simulink model "EV6_LUT_FourWheel_EV6Battery77p4kWh_PowerCorrected"  (R2024a)
settings: Solver=ode4  StartTime=0  StopTime=60  FixedStep=0.001  RelTol=1e-3
PreLoadFcn:
  | VSS_BICYCLE=Simulink.Variant('Dual=0');
  | VSS_DUAL=Simulink.Variant('Dual=1');
  | Dual=1;
  | load('DriveCycle2.mat')
PostLoadFcn:
  | if any(exist('dsrtsu_mdlpostloadfcn', 'file') ~= 0), dsrtsu_mdlpostloadfcn('Execute', bdroot); end
InitFcn:
  | , if any(exist('rtifpga_mdlclblib', 'file') ~= 0), rtifpga_mdlclblib('Init', bdroot); end,
  | , if any(exist('dsmpb_private', 'file') ~= 0), dsmpb_private('dsmpb_mdlclblib', 'Init', bdroot); end,
  | load('DriveCycle2.mat')
model workspace (MAT data in the model file):
  DiffRatio = 10.65
  EV6_2023_BattBranchCapacity_Ah = 55.5236728838
  EV6_2023_BattEnergy_kWh = 77.4
  EV6_2023_BattNominalVoltage_V = 697
  EV6_2023_BattNumCellsParallel = 2
  EV6_2023_BattNumCellsSeries = 192
  EV6_2023_BattOpenVoltCapBpts = [0 0.1 0.2 0.3 0.4 0.5 0.6 0.7 0.8 0.9 1]
  EV6_2023_BattOpenVoltTbl = [2.96762142548 3.40364281191 3.47417488548 3.54470541822 3.61523441014 3.68576186124 3.75628777151 3.82681214095 3.94527005036 4.07101207308 4.2120755254]
  EV6_2023_BattPackCapacity_Ah = 111.047345768
  EV6_2023_BattResistSocBpts = [0 0.2 0.4 0.6 0.8 1]
  EV6_2023_BattResistTbl = [0.0163620057716  0.0172368903217  0.0166967924599  0.0156665372921  0.0190883901835  0.0243044037801; 0.0118174152018  0.0121226074867  0.0102711076249  0.010219317419  0.0111774362286  0.0144365199014; 0.00807187352333  0.00758541551769  0.00750957985901  0.00638499253037  0.00711375471373  0.0083548700057; 0.00375663957972  0.00474065349228  0.00468331433572  0.00455013952048  0.00502364997465  0.00563588419468; 0.00266904525531  0.00337561163613  0.00332012212978  0.00328867807619  0.00355872700708  0.00413211857267; 0.00103635901355  0.00133026843217  0.00127385410071  0.00139778066489  0.00136041773062  0.00187554531454; 0.0019014404175  0.00247483198309  0.00184965021158  0.00284106272499  0.0028595592271  0.00515867444009]
  EV6_2023_BattResistTempBpts = [243.1 253.1 263.1 273.1 283.1 298.1 313.1]
  EV6_2023_InitialPackOCV_V = 726.471714233
  EV6_2023_InitialSOC = 0.638878863672
  EV6_BattCellCapacity_Ah = 60.3
  EV6_BattInitialSOC = 0.638878863672
  EV6_BattOCV_Cell_V = [2.96762142548 3.40364281191 3.47417488548 3.54470541822 3.61523441014 3.68576186124 3.75628777151 3.82681214095 3.94527005036 4.07101207308 4.2120755254]
  EV6_BattOCV_SOC = [0 0.1 0.2 0.3 0.4 0.5 0.6 0.7 0.8 0.9 1]
  EV6_BattPackCapacity_Ah = 120.6
  EV6_BattParallelCells = 2
  EV6_BattResistanceSOC = [0 0.2 0.4 0.6 0.8 1]
  EV6_BattResistanceTable_Ohm = [0.0163620057716  0.0172368903217  0.0166967924599  0.0156665372921  0.0190883901835  0.0243044037801; 0.0118174152018  0.0121226074867  0.0102711076249  0.010219317419  0.0111774362286  0.0144365199014; 0.00807187352333  0.00758541551769  0.00750957985901  0.00638499253037  0.00711375471373  0.0083548700057; 0.00375663957972  0.00474065349228  0.00468331433572  0.00455013952048  0.00502364997465  0.00563588419468; 0.00266904525531  0.00337561163613  0.00332012212978  0.00328867807619  0.00355872700708  0.00413211857267; 0.00103635901355  0.00133026843217  0.00127385410071  0.00139778066489  0.00136041773062  0.00187554531454; 0.0019014404175  0.00247483198309  0.00184965021158  0.00284106272499  0.0028595592271  0.00515867444009]
  EV6_BattResistanceTemp_K = [243.1 253.1 263.1 273.1 283.1 298.1 313.1]
  EV6_BattSeriesCells = 192
  EV6_FinalDriveRatio = 10.65
  EV6_TargetPackResistance_Ohm = 0.132763804608
  Gas = 0.383333333333
undefined symbols (not defined in the file): accel_bp_mps2, AccelCmd, ActTqLF_Nm_, ActTqLR_Nm_, ActTqRF_Nm_, ActTqRR_Nm_, BattChargeLimitMaxPwr, BattChargeLimitSocBpts, BattChargeLimitTbl, BattDischargeLimitSocBpts, BattDischargeLimitTbl, BattDischargeMaxPwr, BrakeMaxPrs, BrakeMaxTrq, ChassisDistCg2FrontAxle, ChassisDistCg2RearAxle, ChassisVehMass, CltchCmd, CoastDown, DecelCmd, DiscIntNeverNeededParam, EnvGravCnst, EnvPrs, EnvTemp, EV6_RegenTorqueGain, EV6_TractionTorqueGain, front_share_regen_3d, front_share_traction_3d, FuelSpecificGrav, GearCmd, h, InitStates, lgSw, limitedMCT, MCT, MtrEffSpdBpts, MtrEffTbl, MtrEffTrqBpts, MtrPwrMax, MtrTrqMax, out_1, pMCT, RealSimPara, Ref_speed, Ref_time, regen_torque_bp_Nm, speed_bp_kph, SteeringCmd, SupvsryCtrlRegenBrkCutOffTbl, SupvsryCtrlRegenSpdBpts, TestScnrioCycleNum, traction_torque_bp_Nm, US06, VEH
libraries: VSIGenLib x65, simulink x54, etargetslib x38, dsmpblib x24, vehdynlibtire x12, autolibshared x11, vehdynlibsuspension x7, vehdynlibtirecommon x7, autolibpowerinfoutils x6, autolibutils x5, autolibsharedcoupling x4, autolibmappedmotor x4
(part 1 of 19)
PreSaveFcn:
  | , if any(exist('dsmpb_private', 'file') ~= 0), dsmpb_private('dsmpb_mdlclblib', 'PreSave', bdroot); end,
CloseFcn:
  | , if any(exist('dsmpb_private', 'file') ~= 0), dsmpb_private('dsmpb_mdlclblib', 'Close', bdroot); end,
settings Model: DataDictionary=DdPassengerEv.sldd  DSMPB_ID_DATA={'18088',struct('BlockId','f88c42c2-e70e-4436-bd85-ff34452e836e','SignalIds',{{'1df572a0-f117-4729-9091-2c1a0a26ec90','0824b86c-995c-4624-95de-4f5a118cf0f7','1af539eb-325a-4e38-9107-84d6b0267392','ebb0fa34-559f-4fe0-b409-8a817ae8753c','d7145080-d35d-4c02-8c9e-cf76ffb14dc2','5075bfde-4142-4aeb-b309-025b37120541','abbab0bd-1456-4252-a37b-ee5f55ea0579','b5d617b8-bb24-4539-9145-e591a0a295f8','7df03788-1936-4801-98c0-dd7f6dfcacba','19949bfb-f246-4995-90e8-29a3751a0fa7','9454b59a-aedd-4270-89a6-1cca43305823','37cf720c-23c2-4b6d-8589-7b035c806643','98db9f76-eafd-4d54-90d2-d997d73b87d4','ff589fc8-5b21-4798-a75e-d26fc35c1fa1','e61b2882-e27e-4f06-b730-5e5281621b34','6605e0e6-8bf3-4a45-a0b0-4b9c1cf463f3','0d0f5161-daad-47a1-bb1d-ec2adbc183ca','48ba6675-0966-4a1c-b127-4f76dca3de94','3c897f11-b2eb-4eb8-b88f-7b7e913c6e41','378f468e-364f-43c5-91f9-fc8ddef6aca6','9c7f20ac-956d-4c19-bdea-31a2a3930ea2','bc252920-9c7c-4b91-a017-ee1d69e3f03c','a5e7a104-8664-4690-a58a-7cbf05737866','fe1cfa34-9b23-4225-85e3-0403f07d36e7','ab40d80a-815e-4994-aacd-e42d283f5b3a','2a4143b2-c438-4d42-997d-0587141eb8f0','2686c37a-8724-40b3-99fb-f8873ba286b8','3707aa1b-88c1-4f14-8f25-f346aa75c252','7413af4b-f834-4020-ad34-3dd98c546e0c','3445835b-9a90-4408-a32d-d76b66b0385b','23c9a144-1259-4fa3-9a16-4a32a7eadff9','5b4206b0-ea89-4111-86f7-7a4fd8c76b72','85c84ea6-72b6-4ccb-9199-727b305580c3','97bb0073-9d03-44a9-972d-49a0eb465678','8c3f0698-b0b6-4624-aa00-3a3096f7cc2f','c968922f-253e-433f-ad46-daf21e902962','21ad150a-19dc-415b-bc1b-b39528ec9221','a3572415-9467-4ff8-a492-c6c1b3cb1b64','700ac678-fb53-40b6-8e97-9eeffe7a1ca8','14ed5f8b-aa1d-402b-b493-5622a729893d','bdbcc0b3-c6a4-485e-8fbf-8c12a8df89e7','7a19cc2b-f06b-466f-ae52-fb8ac6fb0258','87deda6a-2251-4462-8ae0-a20845c776d4','41874d9b-304a-4265-a3a1-69d5c58383ea'}}),'18719',struct('BlockId','79daabbd-4df4-4017-ba65-d977f7e6cd2f','SignalIds',{{'63c99320-3a8a-469e-8a50-5c577229603f'}}),'18720',struct('BlockId','9f21d727-31d5-41b9-aed1-27a40d8edf8b','SignalIds',{{'abab19c9-0d91-46eb-acba-2a4710e305d8'}}),'18721',struct('BlockId','5513e588-accc-447f-8233-209349c29c53','SignalIds',{{'cf7c35a9-6bda-4f5f-bfb5-f51ad44c376b'}}),'18722',struct('BlockId','a427ee23-ff95-4a9c-807f-ad2b61c33ee4','SignalIds',{{'b3e368f1-9670-4dd7-aa42-1fcccca64ddf'}}),'18723',struct('BlockId','53805a71-03ad-4b45-a2ab-66e4ec3700d0','SignalIds',{{'0801da20-d997-46db-8512-e37e1180e77c','d193450d-1a5a-4c8d-a2ac-d5fd306fefe3'}}),'18724',struct('BlockId','4d4909f9-4869-4ae2-8541-060fc5e29366','SignalIds',{{'0588d1ac-5d02-4ce0-9f56-5f4e572c1088','c0609b3e-104e-46bb-beb6-dc1d54d218ce','a0011887-c3f0-4769-95be-c916ccb77447','feb7a80d-e7d1-407d-8b44-49f086fb9d8a'}}),'27205',struct('BlockId','7f292e34-acca-4213-92cf-eac8a4e11745','SignalIds',{{'6a46899f-e089-4ce6-a50d-bdb6920dc331'}}),'27206',struct('BlockId','0e302573-500f-4275-88ba-9cf54fc32ddf','SignalIds',{{'b049b44b-cb75-4882-8bfb-1e055380ad24'}}),'27207',struct('BlockId','894fc26a-3344-4696-abb1-a58f33cf2fe5','SignalIds',{{'56006949-e5f9-49a3-9093-d3c1068f762e'}}),'27282',struct('BlockId','99a4c3a2-8dee-4bd9-95aa-231a7d48a6ad','SignalIds',{{'ad35807f-d183-4bfc-ba2d-784a27a526e2'}}),'27283',struct('BlockId','c3bde5a4-346e-4338-b541-b63d4485ff5c','SignalIds',{{'fd571466-ead4-4f47-b3e3-1d8d73dd83aa'}}),'27284',struct('BlockId','f9cc58a0-b533-4fcd-ba24-c41d1087025b','SignalIds',{{'edc79761-e8e8-4577-bee1-99dd85130da2'}}),'27290',struct('BlockId','912f2a14-bc8b-461e-a925-b64698223e59','SignalIds',{{'776489e0-d1be-4c01-975d-6bf488838e0f'}}),'27291',struct('BlockId','568bb84e-3e6c-4e27-b5f8-f420efc72c29','SignalIds',{{'ed34b8f1-74db-4d36-9a75-d105186c40b5'}}),'27292',struct('BlockId','c169ab68-0334-4d5e-8995-fe0588a530be','SignalIds',{{'fac7e22a-c9c5-48bf-8dd3-1207989a75ce'}}),'27321',struct('BlockId','486c1cde-04a2-4a7b-bb1b-0ecc89f4c4dc','SignalIds',{{'92ff9d42-6575-4421-bf12-cd2858422bf3'}}),'27322',struct('BlockId','3f4e80df-9a0c-4630-abed-705861a8f37f','SignalIds',{{'ecbbb69e-a9c9-45ac-a3ac-ebec06b4c832'}}),'27830',struct('BlockId','3345bd5a-57a2-4283-ba1f-19d9b3e140a9','SignalIds',{{'92c21d5f-d0b1-43b1-b6bc-24cdf5ae3b2f'}}),'27838',struct('BlockId','d4a4d4a9-28f7-4103-93fc-48b8f34cb05d','SignalIds',{{'869cfc04-7b3a-4508-9a04-d408d22a8585','a495f60b-e320-4589-a7da-c9c1e0fb9d66','cadd7efe-3805-4998-94fe-0c2d1fc01ff7','5d968b47-a87d-4eb2-a743-bf289ed725ef','78d13881-677a-4003-a1ce-a7b3fd4b10ed'}}),'27839',struct('BlockId','a8a28146-2bd5-46fa-a2eb-22a81d10cc62','SignalIds',{{'0cba0fcf-c449-40bd-9ed4-ab01110a305a','4e2eaeac-0381-4090-a698-3e33368cf49b'}}),'27843',struct('BlockId','b81313f3-c14d-43f5-aca0-17ec7f04c03a','SignalIds',{{'c33cb8ae-acba-4ded-b0d5-2f0e98182df7'}}),'28333',struct('BlockId','b4192faa-dd44-47ab-a57b-d849e8842c53','SignalIds',{{'3c64dc78-c053-4e1d-a3dc-7d922541f734'}}),'28409',struct('BlockId','364dbf1f-db94-48e0-9add-af905e700009','SignalIds',{{'403b6449-3746-476e-bb2d-b20219d4f4bb','7d755994-2bec-4eab-9fef-7bc71a1fff8b','73ba929b-0017-4bba-a1b8-b6b44c7091ab','1b99e985-b5b3-4b9e-96cf-f375f8e62d9c','ea9d5c72-c4df-42a7-a1b2-83c8aa561c19'}})}  RTICANMMDATA=struct('GeneralSetupData',struct('modelroot','C:\GitDev\Anye\cave_carla_dev\Vehicles\VehicleProjects\Bolt_EV\System','generalsettings',struct('filesettings',struct('destfolder',struct('Name','RTICANMM_FILES','Check',1),'buildfolder',struct('Name','.','Check',1),'AbsDestfolder',struct('Name','C:\GitDev\Anye\cave_carla_dev\Vehicles\VehicleProjects\Bolt_EV\System\RTICANMM_FILES'),'AbsBuildfolder',struct('Name','C:\GitDev\Anye\cave_carla_dev\Vehicles\VehicleProjects\Bolt_EV\System'))),'options',struct('addpaths',1,'rmpaths',1,'addtrcexclusion',true,'cannavigator',struct('checkmonitoring',0),'show_usrtrc',0,'use_usrtrc',0),'advanced',struct('options',ones(1,100)),'MPSetup',{{}},'RTI',struct('Type','DSRT','Ver','4.2p1','Date','11-Feb-2020'),'modelname','CAVE_MachE','block','CAVE_MachE'))  DSRTSU_INTERNAL_RTIFPGA=210  DSRTSU_INTERNAL_RTISTBM_VER=24.1  PauseTimes=45  Creator=9bt  LastModifiedBy=ssl35511
settings SolverCC: AlgebraicLoopSolver=TrustRegion
settings OptimizationCC: BlockReduction=off  ConditionallyExecuteInputs=off  OptimizeBlockIOStorage=off  BufferReuse=off  GlobalBufferReuse=off  ExpressionFolding=off  LocalBlockOutputs=off  OptimizeDataStoreBuffers=off  BusAssignmentInplaceUpdate=off
settings DebuggingCC: MergeDetectMultiDrivingBlocksExec=none  TasksWithSamePriorityMsg=none  ParameterOverflowMsg=none  ParameterUnderflowMsg=error  UnconnectedInputMsg=warning  UnconnectedOutputMsg=warning  UnconnectedLineMsg=warning  UnderSpecifiedDimensionMsg=warning
settings HardwareCC: ProdBitPerLong=64  ProdLargestAtomicInteger=Integer  ProdWordSize=32  ProdHWDeviceType=Custom Processor->Custom
settings ModelReferenceCC: EnableRefExpFcnMdlSchedulingChecks=on  PropagateSignalLabelsOutOfModel=off
settings SFSimCC: MATLABDynamicMemAlloc=off
settings RTWCC: Description=dSPACE Run-Time Target (for VEOS on Windows and ConfigurationDesk)  SystemTargetFile=dsrt.tlc  GenCodeOnly=on  MakeCommand=make_dsrt  TemplateMakefile=dsrt_default_tmf  RTWVerbose=off  GPUComputeCapability=3.5
settings CodeAppCC: MaxIdLength=63  StateflowObjectComments=on
settings STFCustomTargetCC: ParMdlRefBuildCompliant=on  GRTInterface=off  UseToolchainInfoCompliant=off  SystemTargetFile=dsrt.tlc
settings GRTTargetCC: CompOptLevelCompliant=off  ConcurrentExecutionCompliant=off  CombineOutputUpdateFcns=off  MatFileLogging=off  CPPClassGenCompliant=off  UseToolchainInfoCompliant=off

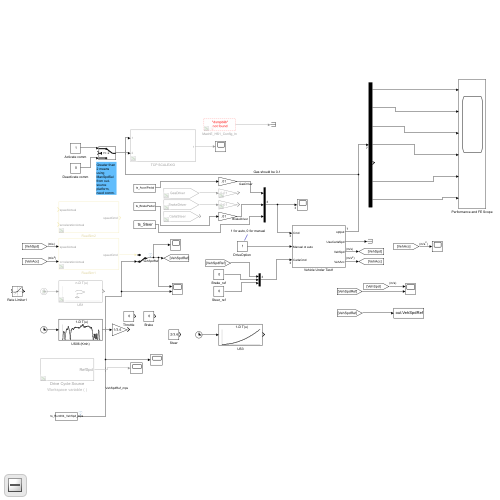
[thumbnail: Simulink's stored preview of the top-level diagram]
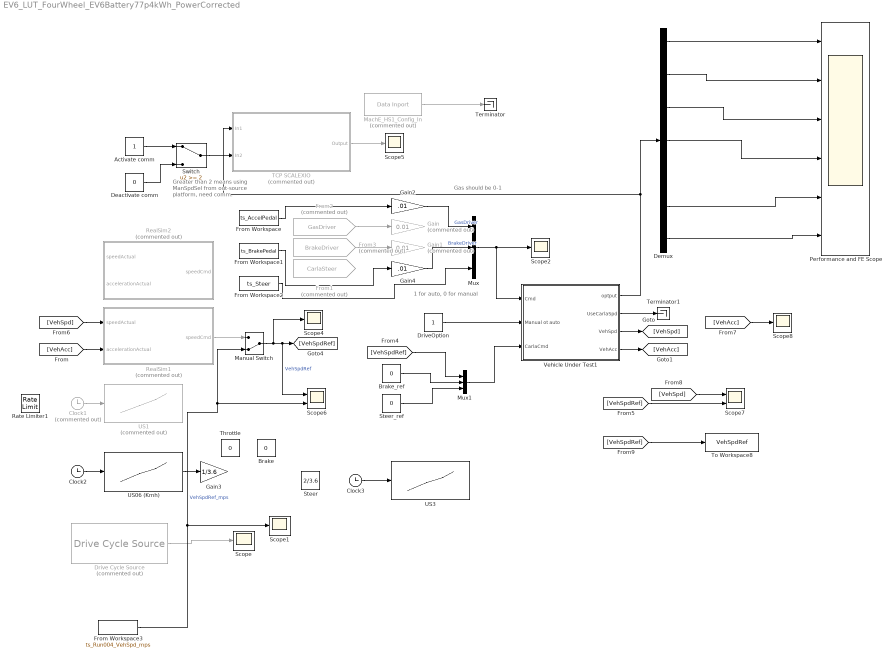
== system EV6_LUT_FourWheel_EV6Battery77p4kWh_PowerCorrected ==
  note: Greater than 2 means using ManSpdSel from out-source platform, need comm.
  note: 1 for auto, 0 for manual
  note: Gas should be 0-1
  Activate comm : Constant
  Brake : Constant  Value=0
  Brake_ref : Constant  Value=0
  Clock1 : Clock  Commented=on
  Clock2 : Clock
  Clock3 : Clock
  Deactivate comm : Constant  Value=0
  Demux : Demux  Outputs=7
  Drive Cycle Source : autolibshared/Drive Cycle Source  Commented=on  cycleVar=Workspace variable  wsVar=spd_kmh_ts  fileVar=cycleFTP75.mat  tfinal=""  cycleRepeat=off  outAccPort=off  outGearPort=off  gearList=No gear data  t_wot1=5  xdot_woto=0  xdot_wot1=30  t_wot2=20  xdot_wot2=0  t_wotend=30  srcUnit=km/h  outUnit=km/h  srcAccUnit=m/s/s  outAccUnit=m/s^2  dt=0  aMode=1  faultOption=off  velBnd=2  velBndUnit=mph  inUnit=m/s  timeBnd=1  failOption=off  stopSim=off  maxFaultCnt=10  maxFaultTime=2  maxTotFaultTime=15  traceOption=off  dtTrace=1  traceWindow=10  lastDCname=Custom Data Set 1  lastOutUnit=mph  lastDT=0  lastTB=1  lastSB=2  forceCalcBound=off
  DriveOption : Constant
  From Workspace : FromWorkspace  VariableName=ts_AccelPedal
  From Workspace1 : FromWorkspace  VariableName=ts_BrakePedal
  From Workspace2 : FromWorkspace  VariableName=ts_Steer
  From Workspace3 : FromWorkspace  VariableName=ts_Run004_VehSpd_mps
  From1 : From  Commented=on  GotoTag=CarlaSteer  TagVisibility=global
  From2 : From  Commented=on  GotoTag=GasDriver  TagVisibility=global
  From3 : From  Commented=on  GotoTag=BrakeDriver  TagVisibility=global
  Gain : Gain  Commented=on  Gain=0.01
  Gain1 : Gain  Commented=on  Gain=0.01
  Gain2 : Gain  Gain=.01
  Gain3 : Gain  Gain=1/3.6
  Gain4 : Gain  Gain=.01
  MachE_HS1_Config_In : dsmpblib/Data Inport  Priority=10000  Commented=on
      settings: SourceProductName=dSPACE Model Interface Package for Simulink (MIPS)
  Manual Switch : ManualSwitch  CurrentSetting=0
  Mux : Mux  Inputs=3
  Mux1 : Mux  Inputs=3
  Performance and FE Scope : Scope  NumInputPorts=6
  Rate Limiter1 : RateLimiter  RisingSlewLimit=4  FallingSlewLimit=-4  SampleTimeMode=inherited
  RealSim1 : Subsystem  Commented=on
  RealSim2 : Subsystem  Commented=on
  Scope{,1..2,4..5,8} (6 alike) : Scope
  Scope6 : Scope  NumInputPorts=2
  Scope7 : Scope  NumInputPorts=2
  Steer : Constant  Value=2/3.6
  Steer_ref : Constant  Value=0
  Switch : Switch  Threshold=2  SaturateOnIntegerOverflow=off  InputSameDT=off
  TCP SCALEXIO : Subsystem  Commented=on
  Terminator : Terminator
  Terminator1 : Terminator
  Throttle : Constant  Value=0
  To Workspace8 : ToWorkspace  VariableName=VehSpdRef  SaveFormat=Timeseries  SampleTime=0.1
  US06 (Kmh) : Lookup_n-D  NumberOfTableDimensions=1  BreakpointsForDimension1=US06.Time  Table=US06.Speed  InternalRulePriority=Speed  RndMeth=Simplest
  US1 : Lookup_n-D  Commented=on  NumberOfTableDimensions=1  BreakpointsForDimension1=out_1.VehSpdRef.Time  Table=out_1.VehSpdRef.Data  InternalRulePriority=Speed  RndMeth=Simplest
  US3 : Lookup_n-D  NumberOfTableDimensions=1  BreakpointsForDimension1=0:1:100  Table=1/100*[0:1:100].^2  InternalRulePriority=Speed  RndMeth=Simplest
  Vehicle Under Test1 : Subsystem
  wires:
  Mux/1 -> Vehicle Under Test1/1(Cmd), Scope2/1
  DriveOption/1 -> Vehicle Under Test1/2(Manual ot auto)
  From2/1 -> Gain/1
  From3/1 -> Gain1/1
  MachE_HS1_Config_In/1 -> Terminator/1
  Vehicle Under Test1/1(optput) -> TCP SCALEXIO/1(In1), Demux/1
  Switch/1 -> TCP SCALEXIO/2(In2)
  TCP SCALEXIO/1(Output) -> Scope5/1
  Deactivate comm/1 -> Switch/3
  Activate comm/1 -> Switch/1
  Manual Switch/1 -> Scope4/1, Scope6/1, [VehSpdRef]  "VehSpdRef"
  RealSim1/1(speedCmd) -> Manual Switch/1
  [VehAcc] -> RealSim1/2(accelerationActual)
  [VehSpd] -> RealSim1/1(speedActual)
  [VehSpdRef] -> Mux1/1
  Mux1/1 -> Vehicle Under Test1/3(CarlaCmd)
  Vehicle Under Test1/3(VehSpd) -> [VehSpd]
  Vehicle Under Test1/4(VehAcc) -> [VehAcc]
  Steer_ref/1 -> Mux1/3
  Brake_ref/1 -> Mux1/2
  Vehicle Under Test1/2(UseCarlaSpd) -> Terminator1/1
  Clock1/1 -> US1/1
  [VehSpdRef] -> Scope7/2
  Demux/1 -> Performance and FE Scope/1
  Demux/7 -> Performance and FE Scope/6
  Demux/6 -> Performance and FE Scope/5
  Demux/4 -> Performance and FE Scope/4
  Demux/3 -> Performance and FE Scope/3
  Demux/2 -> Performance and FE Scope/2
  [VehAcc] -> Scope8/1
  [VehSpd] -> Scope7/1
  [VehSpdRef] -> To Workspace8/1
  Clock2/1 -> US06 (Kmh)/1
  Clock3/1 -> US3/1
  Drive Cycle Source/1 -> Scope/1
  US06 (Kmh)/1 -> Gain3/1
  From Workspace3/1 -> Scope1/1, Scope6/2, Manual Switch/2  "VehSpdRef_mps"
  From Workspace/1 -> Gain2/1
  Gain2/1 -> Mux/1  "GasDriver"
  From Workspace1/1 -> Gain4/1
  Gain4/1 -> Mux/2  "BrakeDriver"
  From Workspace2/1 -> Mux/3

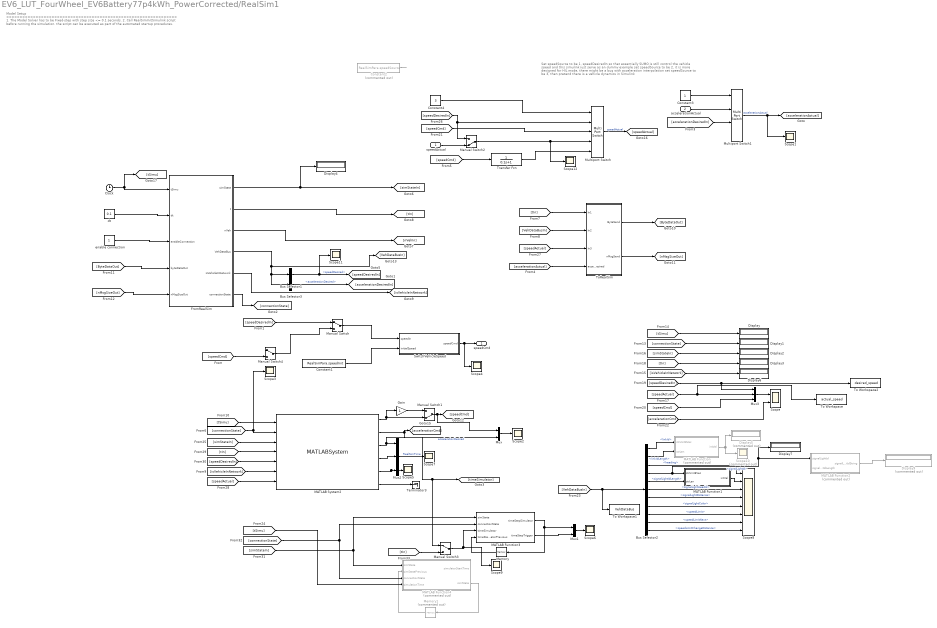
== system EV6_LUT_FourWheel_EV6Battery77p4kWh_PowerCorrected/RealSim1 ==
  note: Set speedSource to be 1, speedDesiredIn so that essentially SUMO is still control the vehicle speed and this simulink just serve as an dummy example
      |
      | set speedSource to be 2, it is more designed for HIL mode, there might be a bug with acceleration interpolation
      |
      | set speedSource to be 3, then pretend there is a vehicle dynamics in Simulink
  note: Model Setup
      | ================================================================
      | 1. The Model Solver has to be Fixed-step with step size <= 0.1 seconds.
      | 2. Call RealSimInitSimulink script before running the simulation. the script can be executed as part of the automated startup procedures.
  speedActual : Inport
  accelerationActual : Inport  Port=2
  Bus Selector1 : BusSelector  OutputSignals=speedDesired
  Bus Selector2 : BusSelector  OutputSignals=linkId,linkIdLength,heading,signalLightId,signalLightIdLength,signalLightHeadId,signalLightDistance,signalLightColor,speedLimit,speedLimitNext,speedLimitChangeDistance
  Bus Selector3 : BusSelector  OutputSignals=accelerationDesired
  Clock : Clock
  Constant1 : Constant  Value=RealSimPara.speedInit
  Constant2 : Constant  Commented=on  Value=RealSimPara.speedSource
  Constant3 : Constant
  Constant4 : Constant  Value=3
  Display{,1..4,6..7} (7 alike) : Display
  Display5 : Display  Commented=on
  Display9 : Display  Commented=on
  FromRealSim : Subsystem
  Gain : Gain
  MATLAB Function : MATLAB Function  Commented=on  TreatAsAtomicUnit=on
  MATLAB Function1 : MATLAB Function  TreatAsAtomicUnit=on
  MATLAB Function2 : MATLAB Function  Commented=on  TreatAsAtomicUnit=on  SystemSampleTime=0.001
  MATLAB Function3 : MATLAB Function  TreatAsAtomicUnit=on
  MATLAB Function4 : MATLAB Function  Commented=on  TreatAsAtomicUnit=on
  MATLAB System2 : MATLABSystem  System=RealSimInterpSpeed  initialSpeed=RealSimPara.speedInit  speedLookAheadHorizon=RealSimPara.tLookahead  speedUpperBound=30  smoothWindow=RealSimPara.smoothWindow  SimulateUsing=Interpreted execution
      mask Type: RealSimInterpSpeed
      mask Display:
      | disp('RealSimInterpSpeed');
      | port_label('input',1,'simulationTime');
      | port_label('input',2,'connectionState');
      | port_label('input',3,'simState');
      | port_label('input',4,'timeReceive');
      | port_label('input',5,'speedReceive');
      | port_label('input',6,'isVehicleInNetwork');
      | port_label('input',7,'speedActual');
      | port_label('output',1,'speedLookAhead');
      | port_label('output',2,'accelerationDesired');
      | port_label('output',3,'timeSimulator');
      | port_label('output',4,'timeStepSimulator');
      | port_label('output',5,'timeStepTrigger');
      | port_label('output',6,'RealSimDelay');
  Manual Switch : ManualSwitch
  Manual Switch1 : ManualSwitch  CurrentSetting=0
  Manual Switch2 : ManualSwitch  CurrentSetting=0
  Manual Switch3 : ManualSwitch
  Manual Switch4 : ManualSwitch
  Memory : Memory
  Memory1 : Memory  Commented=on
  Multiport Switch : MultiPortSwitch  Inputs=4  SaturateOnIntegerOverflow=off  InputSameDT=off
  Multiport Switch1 : MultiPortSwitch  SaturateOnIntegerOverflow=off  InputSameDT=off
  Mux : Mux  Inputs=2
  Mux1 : Mux  Inputs=2
  Mux2 : Mux  Inputs=3
  Mux3 : Mux  Inputs=3
  Scope : Scope  NumInputPorts=2
  Scope{1..7,9,11..12} (10 alike) : Scope
  Scope10 : Scope  Commented=on
  Scope8 : Scope  NumInputPorts=8
  SwitchVehicleSpeed : Subsystem
  Terminator3 : Terminator
  To Workspace : ToWorkspace  VariableName=actual_speed  SaveFormat=Timeseries  SampleTime=0.1
  To Workspace1 : ToWorkspace  VariableName=VehDataBus  SaveFormat=Timeseries  SampleTime=-1
  To Workspace2 : ToWorkspace  VariableName=desired_speed  SaveFormat=Timeseries  SampleTime=0.1
  ToRealSim : Subsystem
  Transfer Fcn : TransferFcn  Denominator=[0.1 1]
  dt : Constant  Value=0.1
  enable connection : Constant
  speedCmd : Outport
  wires:
  [speedCmd] -> Manual Switch4/2
  Manual Switch3/1 -> Scope9/1, MATLAB Function3/3(timeSimulator)
  [tIn] -> Manual Switch3/2
  MATLAB Function4/2(simState) -> Memory1/1
  Memory1/1 -> MATLAB Function4/2(simStatePrevious)
  MATLAB Function3/2(timeStepTrigger) -> Mux1/2
  Mux1/1 -> Scope6/1
  Memory/1 -> MATLAB Function3/4(timeStepSimulatorPrevious)
  MATLAB Function3/1(timeStepSimulator) -> Memory/1, Mux1/1
  [simStateIn] -> MATLAB Function3/1(simState), MATLAB Function4/1("simState ")
  [connectionState] -> MATLAB Function3/2(connectionState), MATLAB Function4/3(connectionState)
  [tSimu] -> MATLAB Function4/4(simulationTime)
  Transfer Fcn/1 -> Multiport Switch/5
  [speedCmd] -> Transfer Fcn/1
  speedActual/1 -> Manual Switch2/2
  Mux/1 -> Scope2/1
  FromRealSim/6(connectionState) -> [connectionState]
  Multiport Switch1/1 -> [accelerationActual], Scope1/1  "accelerationActual"
  accelerationActual/1 -> Multiport Switch1/2
  [accelerationDesiredIn] -> Multiport Switch1/3
  Constant3/1 -> Multiport Switch1/1
  Bus Selector3/1 -> [accelerationDesiredIn]  "<accelerationDesired>"
  Manual Switch/1 -> SwitchVehicleSpeed/1(speedIn)
  SwitchVehicleSpeed/1(speedCmd) -> speedCmd/1, Scope4/1
  Constant1/1 -> SwitchVehicleSpeed/2(initialSpeed)
  [speedDesiredIn] -> Manual Switch/1
  Manual Switch4/1 -> Manual Switch/2
  Constant2/1 -> ?
  ? -> MATLAB Function2/2(signalLightIdLength)
  [simStateIn] -> Display2/1
  Mux3/1 -> Scope/1
  [isVehicleInNetwork] -> MATLAB System2/6
  Bus Selector2/3 -> Scope8/1  "<heading>"
  MATLAB Function1/1(intVal) -> Scope8/2
  ToRealSim/1(ByteSend) -> [ByteDataOut]
  [accelerationActual] -> ToRealSim/4(accelerationDesired)
  Bus Selector2/6 -> Scope8/3  "<signalLightHeadId>"
  Multiport Switch/1 -> [speedActual]  "speedActual"
  [VehDataBusIn] -> ToRealSim/2(In2)
  [accelerationCmd] -> Scope/2
  FromRealSim/5(isVehicleInNetwork) -> [isVehicleInNetwork]
  FromRealSim/2(t) -> [tIn]
  [speedActual] -> ToRealSim/3(In3)
  FromRealSim/1(simState) -> [simStateIn], Display4/1
  ToRealSim/2(nMsgSend) -> [nMsgSizeOut]
  Manual Switch1/1 -> [speedCmd], Mux/1
  Constant4/1 -> Multiport Switch/1
  [speedCmd] -> Mux3/3
  [tIn] -> MATLAB System2/4
  Bus Selector2/2 -> MATLAB Function/2(strLen)  "<linkIdLength>"
  MATLAB Function2/1(signalLightIdString) -> Display9/1
  MATLAB System2/2 -> Mux/2, [accelerationCmd]  "accelerationDesired"
  [tIn] -> ToRealSim/1(In1)
  Bus Selector2/1 -> MATLAB Function/1(strUint8Vec)  "<linkId>"
  MATLAB System2/6 -> Terminator3/1
  [connectionState] -> MATLAB System2/2, Scope3/1
  Manual Switch2/1 -> Multiport Switch/4, Scope12/1
  Bus Selector2/8 -> Scope8/5  "<signalLightColor>"
  MATLAB System2/4 -> Mux2/2
  Bus Selector2/7 -> Scope8/4  "<signalLightDistance>"
  [tIn] -> Display3/1
  Clock/1 -> [tSimu], FromRealSim/1(tSimu)
  [connectionState] -> Display1/1
  [speedActual] -> Mux3/2, To Workspace/1
  FromRealSim/3(nVeh) -> [nVehIn]
  [speedActual] -> MATLAB System2/7
  [speedDesiredIn] -> Multiport Switch/2, Manual Switch2/1
  Bus Selector2/11 -> Scope8/8  "<speedLimitChangeDistance>"
  [nMsgSizeOut] -> FromRealSim/5(nMsgSizeOut)
  [speedDesiredIn] -> MATLAB System2/5
  MATLAB Function/1(intVal) -> Display5/1, Scope10/1
  enable connection/1 -> FromRealSim/3(enableConnection)
  FromRealSim/4(VehDataBus) -> [VehDataBusIn], Bus Selector1/1, Bus Selector3/1
  Bus Selector2/10 -> Scope8/7  "<speedLimitNext>"
  dt/1 -> FromRealSim/2(dt)
  MATLAB System2/3 -> Mux2/1, Manual Switch3/1, [timeSimulator]
  Bus Selector2/4 -> MATLAB Function1/1(strUint8Vec), MATLAB Function2/1(signalLightId), Display7/1  "<signalLightId>"
  [speedDesiredIn] -> Mux3/1, To Workspace2/1
  Bus Selector2/9 -> Scope8/6  "<speedLimit>"
  Bus Selector1/1 -> [speedDesiredIn], Scope11/1  "<speedDesired>"
  Gain/1 -> Manual Switch1/1
  [tSimu] -> MATLAB System2/1
  Mux2/1 -> Scope7/1  "RealSimTime"
  [speedCmd] -> Multiport Switch/3
  MATLAB System2/1 -> Manual Switch1/2, Gain/1
  [VehDataBusIn] -> Bus Selector2/1, To Workspace1/1
  MATLAB System2/5 -> Mux2/3, Scope5/1
  [ByteDataOut] -> FromRealSim/4(byteDataOut)
  [isVehicleInNetwork] -> Display6/1
  [simStateIn] -> MATLAB System2/3
  Bus Selector2/5 -> MATLAB Function1/2(strLen)  "<signalLightIdLength>"
  [tSimu] -> Display/1

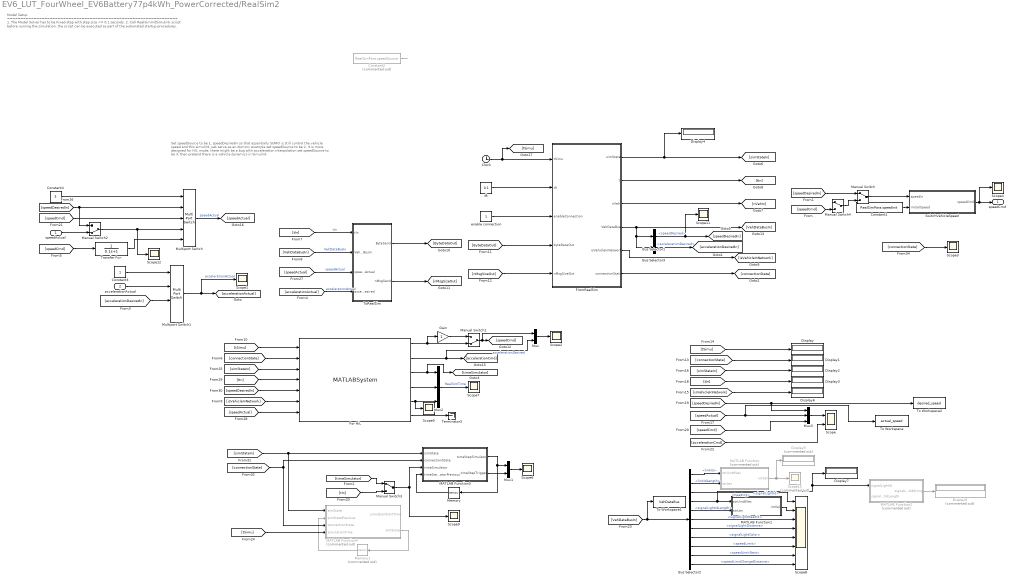
== system EV6_LUT_FourWheel_EV6Battery77p4kWh_PowerCorrected/RealSim2 ==
  note: Set speedSource to be 1, speedDesiredIn so that essentially SUMO is still control the vehicle speed and this simulink just serve as an dummy example
      |
      | set speedSource to be 2, it is more designed for HIL mode, there might be a bug with acceleration interpolation
      |
      | set speedSource to be 3, then pretend there is a vehicle dynamics in Simulink
  note: Model Setup
      | ================================================================
      | 1. The Model Solver has to be Fixed-step with step size <= 0.1 seconds.
      | 2. Call RealSimInitSimulink script before running the simulation. the script can be executed as part of the automated startup procedures.
  speedActual : Inport
  accelerationActual : Inport  Port=2
  Bus Selector1 : BusSelector  OutputSignals=speedDesired
  Bus Selector2 : BusSelector  OutputSignals=linkId,linkIdLength,heading,signalLightId,signalLightIdLength,signalLightHeadId,signalLightDistance,signalLightColor,speedLimit,speedLimitNext,speedLimitChangeDistance
  Bus Selector3 : BusSelector  OutputSignals=accelerationDesired
  Clock : Clock
  Constant1 : Constant  Value=RealSimPara.speedInit
  Constant2 : Constant  Commented=on  Value=RealSimPara.speedSource
  Constant3 : Constant
  Constant4 : Constant  Value=3
  Display{,1..4,6..7} (7 alike) : Display
  Display5 : Display  Commented=on
  Display9 : Display  Commented=on
  For HiL : MATLABSystem  System=RealSimInterpSpeed  initialSpeed=RealSimPara.speedInit  speedLookAheadHorizon=RealSimPara.tLookahead  speedUpperBound=30  smoothWindow=RealSimPara.smoothWindow  SimulateUsing=Interpreted execution
      mask Type: RealSimInterpSpeed
      mask Display:
      | disp('RealSimInterpSpeed');
      | port_label('input',1,'simulationTime');
      | port_label('input',2,'connectionState');
      | port_label('input',3,'simState');
      | port_label('input',4,'timeReceive');
      | port_label('input',5,'speedReceive');
      | port_label('input',6,'isVehicleInNetwork');
      | port_label('input',7,'speedActual');
      | port_label('output',1,'speedLookAhead');
      | port_label('output',2,'accelerationDesired');
      | port_label('output',3,'timeSimulator');
      | port_label('output',4,'timeStepSimulator');
      | port_label('output',5,'timeStepTrigger');
      | port_label('output',6,'RealSimDelay');
  FromRealSim : Subsystem
  Gain : Gain
  MATLAB Function : MATLAB Function  Commented=on  TreatAsAtomicUnit=on
  MATLAB Function1 : MATLAB Function  TreatAsAtomicUnit=on
  MATLAB Function2 : MATLAB Function  Commented=on  TreatAsAtomicUnit=on  SystemSampleTime=0.001
  MATLAB Function3 : MATLAB Function  TreatAsAtomicUnit=on
  MATLAB Function4 : MATLAB Function  Commented=on  TreatAsAtomicUnit=on
  Manual Switch : ManualSwitch
  Manual Switch1 : ManualSwitch  CurrentSetting=0
  Manual Switch2 : ManualSwitch  CurrentSetting=0
  Manual Switch3 : ManualSwitch
  Manual Switch4 : ManualSwitch
  Memory : Memory
  Memory1 : Memory  Commented=on
  Multiport Switch : MultiPortSwitch  Inputs=4  SaturateOnIntegerOverflow=off  InputSameDT=off
  Multiport Switch1 : MultiPortSwitch  SaturateOnIntegerOverflow=off  InputSameDT=off
  Mux : Mux  Inputs=2
  Mux1 : Mux  Inputs=2
  Mux2 : Mux  Inputs=3
  Mux3 : Mux  Inputs=3
  Scope : Scope  NumInputPorts=2
  Scope{1..7,9,11..12} (10 alike) : Scope
  Scope10 : Scope  Commented=on
  Scope8 : Scope  NumInputPorts=8
  SwitchVehicleSpeed : Subsystem
  Terminator3 : Terminator
  To Workspace : ToWorkspace  VariableName=actual_speed  SaveFormat=Timeseries  SampleTime=0.1
  To Workspace1 : ToWorkspace  VariableName=VehDataBus  SaveFormat=Timeseries  SampleTime=-1
  To Workspace2 : ToWorkspace  VariableName=desired_speed  SaveFormat=Timeseries  SampleTime=0.1
  ToRealSim : Subsystem
  Transfer Fcn : TransferFcn  Denominator=[0.1 1]
  dt : Constant  Value=0.1
  enable connection : Constant
  speedCmd : Outport
  wires:
  [speedCmd] -> Manual Switch4/2
  Manual Switch3/1 -> MATLAB Function3/3(timeSimulator), Scope9/1
  [tIn] -> Manual Switch3/2
  MATLAB Function4/2(simState) -> Memory1/1
  Memory1/1 -> MATLAB Function4/2(simStatePrevious)
  MATLAB Function3/2(timeStepTrigger) -> Mux1/2
  Mux1/1 -> Scope6/1
  Memory/1 -> MATLAB Function3/4(timeStepSimulatorPrevious)
  MATLAB Function3/1(timeStepSimulator) -> Memory/1, Mux1/1
  [simStateIn] -> MATLAB Function4/1("simState "), MATLAB Function3/1(simState)
  [connectionState] -> MATLAB Function3/2(connectionState), MATLAB Function4/3(connectionState)
  [tSimu] -> MATLAB Function4/4(simulationTime)
  Transfer Fcn/1 -> Multiport Switch/5
  [speedCmd] -> Transfer Fcn/1
  speedActual/1 -> Manual Switch2/2
  Mux/1 -> Scope2/1
  FromRealSim/6(connectionState) -> [connectionState]
  Multiport Switch1/1 -> [accelerationActual], Scope1/1  "accelerationActual"
  accelerationActual/1 -> Multiport Switch1/2
  [accelerationDesiredIn] -> Multiport Switch1/3
  Constant3/1 -> Multiport Switch1/1
  Bus Selector3/1 -> [accelerationDesiredIn]  "<accelerationDesired>"
  Manual Switch/1 -> SwitchVehicleSpeed/1(speedIn)
  SwitchVehicleSpeed/1(speedCmd) -> speedCmd/1, Scope4/1
  Constant1/1 -> SwitchVehicleSpeed/2(initialSpeed)
  [speedDesiredIn] -> Manual Switch/1
  Manual Switch4/1 -> Manual Switch/2
  Constant2/1 -> ?
  [simStateIn] -> Display2/1
  Mux3/1 -> Scope/1
  [isVehicleInNetwork] -> For HiL/6
  Bus Selector2/3 -> Scope8/1  "<heading>"
  MATLAB Function1/1(intVal) -> Scope8/2
  ToRealSim/1(ByteSend) -> [ByteDataOut]
  [accelerationActual] -> ToRealSim/4(accelerationDesired)  "accelerationActual"
  Bus Selector2/6 -> Scope8/3  "<signalLightHeadId>"
  Multiport Switch/1 -> [speedActual]  "speedActual"
  [VehDataBusIn] -> ToRealSim/2(VehDataBusIn)  "VehDataBusIn"
  [accelerationCmd] -> Scope/2
  FromRealSim/5(isVehicleInNetwork) -> [isVehicleInNetwork]
  FromRealSim/2(t) -> [tIn]
  [speedActual] -> ToRealSim/3(speedActual)  "speedActual"
  FromRealSim/1(simState) -> [simStateIn], Display4/1
  ToRealSim/2(nMsgSend) -> [nMsgSizeOut]
  Manual Switch1/1 -> [speedCmd], Mux/1
  Constant4/1 -> Multiport Switch/1
  [speedCmd] -> Mux3/3
  [tIn] -> For HiL/4
  Bus Selector2/2 -> MATLAB Function/2(strLen)  "<linkIdLength>"
  MATLAB Function2/1(signalLightIdString) -> Display9/1
  For HiL/2 -> Mux/2, [accelerationCmd]  "accelerationDesired"
  [tIn] -> ToRealSim/1(tIn)  "tIn"
  Bus Selector2/1 -> MATLAB Function/1(strUint8Vec)  "<linkId>"
  For HiL/6 -> Terminator3/1
  [connectionState] -> For HiL/2
  Manual Switch2/1 -> Multiport Switch/4, Scope12/1
  Bus Selector2/8 -> Scope8/5  "<signalLightColor>"
  For HiL/4 -> Mux2/2
  Bus Selector2/7 -> Scope8/4  "<signalLightDistance>"
  [tIn] -> Display3/1
  Clock/1 -> [tSimu], FromRealSim/1(tSimu)
  [connectionState] -> Display1/1
  [speedActual] -> Mux3/2, To Workspace/1
  FromRealSim/3(nVeh) -> [nVehIn]
  [speedActual] -> For HiL/7
  [speedDesiredIn] -> Multiport Switch/2, Manual Switch2/1
  Bus Selector2/11 -> Scope8/8  "<speedLimitChangeDistance>"
  [nMsgSizeOut] -> FromRealSim/5(nMsgSizeOut)
  [speedDesiredIn] -> For HiL/5
  MATLAB Function/1(intVal) -> Scope10/1, Display5/1
  enable connection/1 -> FromRealSim/3(enableConnection)
  FromRealSim/4(VehDataBus) -> [VehDataBusIn], Bus Selector1/1, Bus Selector3/1
  Bus Selector2/10 -> Scope8/7  "<speedLimitNext>"
  dt/1 -> FromRealSim/2(dt)
  For HiL/3 -> [timeSimulator], Mux2/1
  Bus Selector2/4 -> MATLAB Function1/1(strUint8Vec), MATLAB Function2/1(signalLightId), Display7/1  "<signalLightId>"
  [speedDesiredIn] -> Mux3/1, To Workspace2/1
  Bus Selector2/9 -> Scope8/6  "<speedLimit>"
  Bus Selector1/1 -> [speedDesiredIn], Scope11/1  "<speedDesired>"
  Gain/1 -> Manual Switch1/1
  [tSimu] -> For HiL/1
  Mux2/1 -> Scope7/1  "RealSimTime"
  [speedCmd] -> Multiport Switch/3
  For HiL/1 -> Gain/1, Manual Switch1/2
  [VehDataBusIn] -> To Workspace1/1, Bus Selector2/1
  For HiL/5 -> Mux2/3, Scope5/1
  [ByteDataOut] -> FromRealSim/4(byteDataOut)
  [isVehicleInNetwork] -> Display6/1
  [simStateIn] -> For HiL/3
  Bus Selector2/5 -> MATLAB Function1/2(strLen)  "<signalLightIdLength>"
  [tSimu] -> Display/1
  [timeSimulator] -> Manual Switch3/1
  [connectionState] -> Scope3/1

== system EV6_LUT_FourWheel_EV6Battery77p4kWh_PowerCorrected/TCP SCALEXIO ==
  note: Receiving gas, brake, steering; or three identical speeds
  note: Sending out x, y, heading, time, and speed
  In1 : Inport
  In2 : Inport  Port=2
  Constant2 : Constant  Value=zeros(1004,1);  OutDataTypeStr=uint8
  Data Type Conversion1 : DataTypeConversion  OutDataTypeStr=double  SaturateOnIntegerOverflow=off  RndMeth=Floor
  Data Type Conversion2 : DataTypeConversion  SaturateOnIntegerOverflow=off  RndMeth=Floor
  Data Type Conversion3 : DataTypeConversion  OutDataTypeStr=boolean  SaturateOnIntegerOverflow=off  RndMeth=Floor
  Defloater{,1..4} (5 alike) : VSIGenLib/Defloater  SystemSampleTime=-1  VariantActivationTime=update diagram  AllowFlexibleInterface=on  Latency=0  AutoFrameSizeCalculation=off
  Demux{,2..5} (5 alike) : Demux
  Demux1 : Demux  Outputs=5
  Display3 : Display
  Ethernet Setup Carla : dsmpblib/Data Inport  Priority=10000
      settings: SourceProductName=dSPACE Model Interface Package for Simulink (MIPS)
  Floater : VSIGenLib/Floater  SystemSampleTime=-1  VariantActivationTime=update diagram  AllowFlexibleInterface=on  Latency=0  AutoFrameSizeCalculation=off
  Floater1 : VSIGenLib/Floater  SystemSampleTime=-1  VariantActivationTime=update diagram  AllowFlexibleInterface=on  Latency=0  AutoFrameSizeCalculation=off
  Floater2 : VSIGenLib/Floater  SystemSampleTime=-1  VariantActivationTime=update diagram  AllowFlexibleInterface=on  Latency=0  AutoFrameSizeCalculation=off
  Mux : Mux  Inputs=21
  Mux1 : Mux  Inputs=3
  Receive [TCP Carla] : dsmpblib/Data Inport  Priority=10000
      settings: SourceProductName=dSPACE Model Interface Package for Simulink (MIPS)
  Scope1 : Scope
  Scope4 : Scope
  Selector1 : Selector  InputPortWidth=1024  IndexOptions=Index vector (dialog)  Indices=[8 7 6 5]  OutputSizes=1
  Selector2 : Selector  InputPortWidth=1024  IndexOptions=Index vector (dialog)  Indices=[12 11 10 9]  OutputSizes=1
  Selector4 : Selector  InputPortWidth=1024  IndexOptions=Index vector (dialog)  Indices=[4 3 2 1]  OutputSizes=1
  SpdAdjust : Gain  Gain=1.1414
  Status/Control_In [TCP Carla] : dsmpblib/Data Inport  Priority=10000
      settings: SourceProductName=dSPACE Model Interface Package for Simulink (MIPS)
  Status/Control_Out [TCP Carla] : dsmpblib/Data Outport  Priority=-10000
      settings: SourceProductName=dSPACE Model Interface Package for Simulink (MIPS)
  Terminator{1..5} (5 alike) : Terminator
  Transmit_In [TCP Carla] : dsmpblib/Data Inport  Priority=10000
      settings: SourceProductName=dSPACE Model Interface Package for Simulink (MIPS)
  Transmit_Out [TCP Carla] : dsmpblib/Data Outport  Priority=-10000
      settings: SourceProductName=dSPACE Model Interface Package for Simulink (MIPS)
  uint8 (unsigned 8) 4 : etargetslib/Byte Pack  datatypes={'uint8'}  byteAlign=1
  Output : Outport
  wires:
  Demux4/4 -> Mux/16
  Demux3/4 -> Mux/12
  Defloater1/1 -> Demux2/1
  Mux/1 -> Data Type Conversion2/1
  Demux4/2 -> Mux/14
  Demux3/1 -> Mux/9
  Demux/4 -> Mux/4
  Demux/1 -> Mux/1
  Demux2/4 -> Mux/8
  Demux1/3 -> Defloater2/1
  Defloater/1 -> Demux/1
  Defloater3/1 -> Demux4/1
  Demux3/3 -> Mux/11
  Demux1/2 -> Defloater1/1
  Demux2/2 -> Mux/6
  Constant2/1 -> uint8 (unsigned 8) 4/1
  Demux1/1 -> Defloater/1
  Defloater2/1 -> Demux3/1
  Demux1/4 -> Defloater3/1
  Demux3/2 -> Mux/10
  Demux/3 -> Mux/3
  Demux/2 -> Mux/2
  In1/1 -> Demux1/1
  Demux2/1 -> Mux/5
  Demux4/1 -> Mux/13
  Demux2/3 -> Mux/7
  Demux4/3 -> Mux/15
  Data Type Conversion2/1 -> Transmit_Out [TCP Carla]/1
  Transmit_In [TCP Carla]/2 -> Terminator2/1
  Transmit_In [TCP Carla]/1 -> Terminator1/1
  Receive [TCP Carla]/1 -> Selector4/1, Selector2/1, Selector1/1
  Selector4/1 -> Floater/1
  Floater/1 -> Display3/1, Mux1/1
  Receive [TCP Carla]/2 -> Terminator4/1
  Data Type Conversion3/1 -> Status/Control_Out [TCP Carla]/1
  In2/1 -> Data Type Conversion3/1
  Receive [TCP Carla]/4 -> Terminator5/1
  Receive [TCP Carla]/3 -> Terminator3/1
  Status/Control_In [TCP Carla]/1 -> Scope4/1
  Ethernet Setup Carla/1 -> Scope1/1
  Demux1/5 -> SpdAdjust/1
  Defloater4/1 -> Demux5/1
  Demux5/2 -> Mux/18
  Demux5/3 -> Mux/19
  Demux5/4 -> Mux/20
  uint8 (unsigned 8) 4/1 -> Mux/21
  Demux5/1 -> Mux/17
  SpdAdjust/1 -> Defloater4/1
  Selector1/1 -> Floater1/1
  Mux1/1 -> Data Type Conversion1/1
  Floater1/1 -> Mux1/2
  Selector2/1 -> Floater2/1
  Floater2/1 -> Mux1/3
  Data Type Conversion1/1 -> Output/1
